simulink model "V2GCKT"  (R2016b)
settings: Solver=ode23t  StartTime=0.0  StopTime=1  RelTol=1e-3
undefined symbols (not defined in the file): Ion, Lithium
libraries: powerlib x27, powerlib_meascontrol x8, simulink x5, electricdrivelib x1
settings Model: Creator=acer  LastModifiedBy=acer

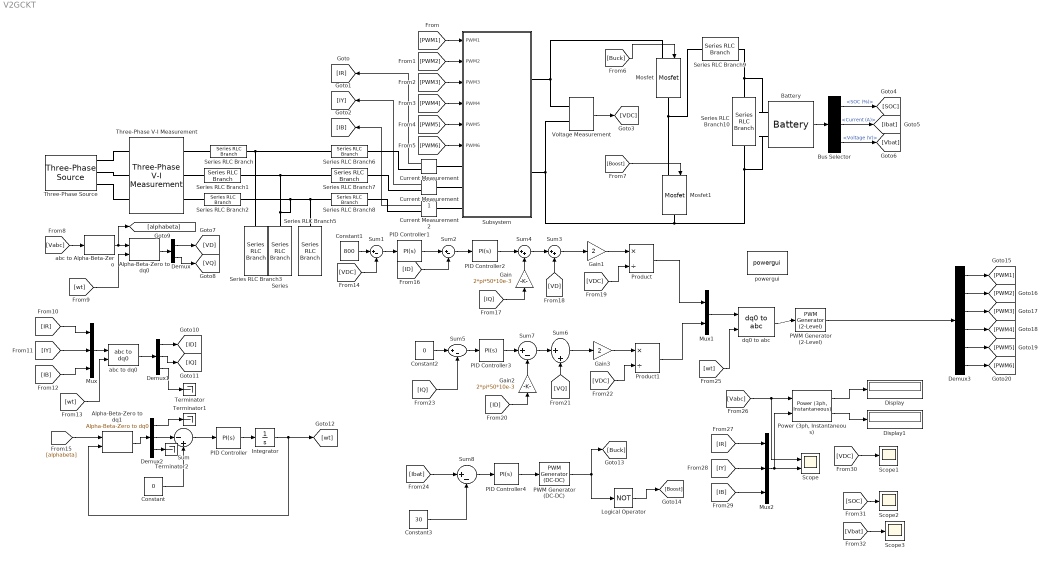
== system V2GCKT ==
  Alpha-Beta-Zero to dq0 : powerlib_meascontrol/Transformations/Alpha-Beta-Zero to dq0  Alignment=90 degrees behind phase A axis
  Alpha-Beta-Zero to dq1 : powerlib_meascontrol/Transformations/Alpha-Beta-Zero to dq0  Alignment=90 degrees behind phase A axis
  Battery : electricdrivelib/Extra Sources/Battery  BatType=Lithium-Ion  ShowTempParam=off  ThermalPreset=no  NomV=360  NomQ=300  SOC=50  Batt_Tr=1  PresetModel=on  MaxQ=300  MinV=270  FullV=419.0354  Dis_rate=130.4348  R=0.012  Normal_OP=271.3043  expZone="[388.9389      14.73913]"  current=[6.5 13 32.5]  Units=Time  Tci=20  NomT=25  T2=0  MaxQ2=2.208  FullV2=3.45  Normal_OP2=2.8  expZone2="[3.22        0.23]"  Rca=0.6  ti=1000  Dp=0
  Bus Selector : BusSelector  OutputSignals=SOC (%),Current (A),Voltage (V)
  Constant : Constant  Value=0
  Constant1 : Constant  Value=800
  Constant2 : Constant  Value=0
  Constant3 : Constant  Value=30
  Current Measurement : powerlib/Measurements/Current Measurement  PhasorSimulation=off  OutputType=Complex  PSBequivalent=0
  Current Measurement1 : powerlib/Measurements/Current Measurement  PhasorSimulation=off  OutputType=Complex  PSBequivalent=0
  Current Measurement2 : powerlib/Measurements/Current Measurement  PhasorSimulation=off  OutputType=Complex  PSBequivalent=0
  Demux : Demux  Outputs=2
  Demux1 : Demux  Outputs=3
  Demux2 : Demux  Outputs=3
  Demux3 : Demux  Outputs=6
  Display : Display
  Display1 : Display
  Gain : Gain  Gain=2*pi*50*10e-3
  Gain1 : Gain  Gain=2
  Gain2 : Gain  Gain=2*pi*50*10e-3
  Gain3 : Gain  Gain=2
  Integrator : Integrator
  Logical Operator : Logic  Operator=NOT  AllPortsSameDT=off  OutDataTypeStr=boolean
  Mosfet : powerlib/Power Electronics/Mosfet  Ron=0.1  Lon=0  Rd=0.01  Vfd=0  IC=0  Rs=1e5  Cs=inf  Measurements=off
  Mosfet1 : powerlib/Power Electronics/Mosfet  Ron=0.1  Lon=0  Rd=0.01  Vfd=0  IC=0  Rs=1e5  Cs=inf  Measurements=off
  Mux : Mux  Inputs=3
  Mux1 : Mux  Inputs=2
  Mux2 : Mux  Inputs=3
  PID Controller : simulink/Continuous/PID Controller  Controller=PI  TimeDomain=Continuous-time  SampleTime=-1  IntegratorMethod=Forward Euler  FilterMethod=Forward Euler  Form=Parallel  UseFilter=on  ControllerParametersSource=internal  P=10  I=50000  D=0  N=100  InitialConditionSource=internal  InitialConditionForIntegrator=0  InitialConditionForFilter=0  ExternalReset=none  LimitOutput=off  UpperSaturationLimit=inf  LowerSaturationLimit=-inf  LinearizeAsGain=on  AntiWindupMode=none  Kb=1  TrackingMode=off  Kt=1  PParamMin=[]  PParamMax=[]  IParamMin=[]  IParamMax=[]  DParamMin=[]  DParamMax=[]  NParamMin=[]  NParamMax=[]  KbParamMin=[]  KbParamMax=[]  KtParamMin=[]  KtParamMax=[]  POutMin=[]  POutMax=[]  IOutMin=[]  IOutMax=[]  DOutMin=[]  DOutMax=[]  NOutMin=[]  NOutMax=[]  KbOutMin=[]  KbOutMax=[]  KtOutMin=[]  KtOutMax=[]  IntegratorOutMin=[]  IntegratorOutMax=[]  FilterOutMin=[]  FilterOutMax=[]  SumOutMin=[]  SumOutMax=[]  SumI1OutMin=[]  SumI1OutMax=[]  SumI2OutMin=[]  SumI2OutMax=[]  SumI3OutMin=[]  SumI3OutMax=[]  SumDOutMin=[]  SumDOutMax=[]  SaturationOutMin=[]  SaturationOutMax=[]  IntegratorContinuousStateAttributes=''  IntegratorStateMustResolveToSignalObject=off  IntegratorRTWStateStorageClass=Auto  FilterContinuousStateAttributes=''  FilterStateMustResolveToSignalObject=off  FilterRTWStateStorageClass=Auto  DifferentiatorICPrevScaledInput=0  DifferentiatorOutMin=[]  DifferentiatorOutMax=[]
  PID Controller1 : simulink/Continuous/PID Controller  Controller=PI  TimeDomain=Continuous-time  SampleTime=-1  IntegratorMethod=Forward Euler  FilterMethod=Forward Euler  Form=Parallel  UseFilter=on  ControllerParametersSource=internal  P=0.5  I=5  D=0  N=100  InitialConditionSource=internal  InitialConditionForIntegrator=0  InitialConditionForFilter=0  ExternalReset=none  LimitOutput=off  UpperSaturationLimit=inf  LowerSaturationLimit=-inf  LinearizeAsGain=on  AntiWindupMode=none  Kb=1  TrackingMode=off  Kt=1  PParamMin=[]  PParamMax=[]  IParamMin=[]  IParamMax=[]  DParamMin=[]  DParamMax=[]  NParamMin=[]  NParamMax=[]  KbParamMin=[]  KbParamMax=[]  KtParamMin=[]  KtParamMax=[]  POutMin=[]  POutMax=[]  IOutMin=[]  IOutMax=[]  DOutMin=[]  DOutMax=[]  NOutMin=[]  NOutMax=[]  KbOutMin=[]  KbOutMax=[]  KtOutMin=[]  KtOutMax=[]  IntegratorOutMin=[]  IntegratorOutMax=[]  FilterOutMin=[]  FilterOutMax=[]  SumOutMin=[]  SumOutMax=[]  SumI1OutMin=[]  SumI1OutMax=[]  SumI2OutMin=[]  SumI2OutMax=[]  SumI3OutMin=[]  SumI3OutMax=[]  SumDOutMin=[]  SumDOutMax=[]  SaturationOutMin=[]  SaturationOutMax=[]  IntegratorContinuousStateAttributes=''  IntegratorStateMustResolveToSignalObject=off  IntegratorRTWStateStorageClass=Auto  FilterContinuousStateAttributes=''  FilterStateMustResolveToSignalObject=off  FilterRTWStateStorageClass=Auto  DifferentiatorICPrevScaledInput=0  DifferentiatorOutMin=[]  DifferentiatorOutMax=[]
  PID Controller2 : simulink/Continuous/PID Controller  Controller=PI  TimeDomain=Continuous-time  SampleTime=-1  IntegratorMethod=Forward Euler  FilterMethod=Forward Euler  Form=Parallel  UseFilter=on  ControllerParametersSource=internal  P=25  I=500  D=0  N=100  InitialConditionSource=internal  InitialConditionForIntegrator=0  InitialConditionForFilter=0  ExternalReset=none  LimitOutput=off  UpperSaturationLimit=inf  LowerSaturationLimit=-inf  LinearizeAsGain=on  AntiWindupMode=none  Kb=1  TrackingMode=off  Kt=1  PParamMin=[]  PParamMax=[]  IParamMin=[]  IParamMax=[]  DParamMin=[]  DParamMax=[]  NParamMin=[]  NParamMax=[]  KbParamMin=[]  KbParamMax=[]  KtParamMin=[]  KtParamMax=[]  POutMin=[]  POutMax=[]  IOutMin=[]  IOutMax=[]  DOutMin=[]  DOutMax=[]  NOutMin=[]  NOutMax=[]  KbOutMin=[]  KbOutMax=[]  KtOutMin=[]  KtOutMax=[]  IntegratorOutMin=[]  IntegratorOutMax=[]  FilterOutMin=[]  FilterOutMax=[]  SumOutMin=[]  SumOutMax=[]  SumI1OutMin=[]  SumI1OutMax=[]  SumI2OutMin=[]  SumI2OutMax=[]  SumI3OutMin=[]  SumI3OutMax=[]  SumDOutMin=[]  SumDOutMax=[]  SaturationOutMin=[]  SaturationOutMax=[]  IntegratorContinuousStateAttributes=''  IntegratorStateMustResolveToSignalObject=off  IntegratorRTWStateStorageClass=Auto  FilterContinuousStateAttributes=''  FilterStateMustResolveToSignalObject=off  FilterRTWStateStorageClass=Auto  DifferentiatorICPrevScaledInput=0  DifferentiatorOutMin=[]  DifferentiatorOutMax=[]
  PID Controller3 : simulink/Continuous/PID Controller  Controller=PI  TimeDomain=Continuous-time  SampleTime=-1  IntegratorMethod=Forward Euler  FilterMethod=Forward Euler  Form=Parallel  UseFilter=on  ControllerParametersSource=internal  P=25  I=500  D=0  N=100  InitialConditionSource=internal  InitialConditionForIntegrator=0  InitialConditionForFilter=0  ExternalReset=none  LimitOutput=off  UpperSaturationLimit=inf  LowerSaturationLimit=-inf  LinearizeAsGain=on  AntiWindupMode=none  Kb=1  TrackingMode=off  Kt=1  PParamMin=[]  PParamMax=[]  IParamMin=[]  IParamMax=[]  DParamMin=[]  DParamMax=[]  NParamMin=[]  NParamMax=[]  KbParamMin=[]  KbParamMax=[]  KtParamMin=[]  KtParamMax=[]  POutMin=[]  POutMax=[]  IOutMin=[]  IOutMax=[]  DOutMin=[]  DOutMax=[]  NOutMin=[]  NOutMax=[]  KbOutMin=[]  KbOutMax=[]  KtOutMin=[]  KtOutMax=[]  IntegratorOutMin=[]  IntegratorOutMax=[]  FilterOutMin=[]  FilterOutMax=[]  SumOutMin=[]  SumOutMax=[]  SumI1OutMin=[]  SumI1OutMax=[]  SumI2OutMin=[]  SumI2OutMax=[]  SumI3OutMin=[]  SumI3OutMax=[]  SumDOutMin=[]  SumDOutMax=[]  SaturationOutMin=[]  SaturationOutMax=[]  IntegratorContinuousStateAttributes=''  IntegratorStateMustResolveToSignalObject=off  IntegratorRTWStateStorageClass=Auto  FilterContinuousStateAttributes=''  FilterStateMustResolveToSignalObject=off  FilterRTWStateStorageClass=Auto  DifferentiatorICPrevScaledInput=0  DifferentiatorOutMin=[]  DifferentiatorOutMax=[]
  PID Controller4 : simulink/Continuous/PID Controller  Controller=PI  TimeDomain=Continuous-time  SampleTime=-1  IntegratorMethod=Forward Euler  FilterMethod=Forward Euler  Form=Parallel  UseFilter=on  ControllerParametersSource=internal  P=0.005  I=10  D=0  N=100  InitialConditionSource=internal  InitialConditionForIntegrator=0  InitialConditionForFilter=0  ExternalReset=none  LimitOutput=on  UpperSaturationLimit=0.95  LowerSaturationLimit=0  LinearizeAsGain=on  AntiWindupMode=none  Kb=1  TrackingMode=off  Kt=1  PParamMin=[]  PParamMax=[]  IParamMin=[]  IParamMax=[]  DParamMin=[]  DParamMax=[]  NParamMin=[]  NParamMax=[]  KbParamMin=[]  KbParamMax=[]  KtParamMin=[]  KtParamMax=[]  POutMin=[]  POutMax=[]  IOutMin=[]  IOutMax=[]  DOutMin=[]  DOutMax=[]  NOutMin=[]  NOutMax=[]  KbOutMin=[]  KbOutMax=[]  KtOutMin=[]  KtOutMax=[]  IntegratorOutMin=[]  IntegratorOutMax=[]  FilterOutMin=[]  FilterOutMax=[]  SumOutMin=[]  SumOutMax=[]  SumI1OutMin=[]  SumI1OutMax=[]  SumI2OutMin=[]  SumI2OutMax=[]  SumI3OutMin=[]  SumI3OutMax=[]  SumDOutMin=[]  SumDOutMax=[]  SaturationOutMin=[]  SaturationOutMax=[]  IntegratorContinuousStateAttributes=''  IntegratorStateMustResolveToSignalObject=off  IntegratorRTWStateStorageClass=Auto  FilterContinuousStateAttributes=''  FilterStateMustResolveToSignalObject=off  FilterRTWStateStorageClass=Auto  DifferentiatorICPrevScaledInput=0  DifferentiatorOutMin=[]  DifferentiatorOutMax=[]
  PWM Generator (2-Level) : powerlib_meascontrol/Pulse & Signal Generators/PWM Generator (2-Level)  ModulatorType=Three-phase bridge (6 pulses)  ModulatorMode=Unsynchronized  Fc=10000  Pc=90  nF=27  MinMax="[ -1  1 ]"  SamplingTechnique=Natural  ModulatingSignals=off  m=0.8  Freq=60  Phase=0  Ts=0  ShowCarrierOutport=off
  PWM Generator (DC-DC) : powerlib_meascontrol/Pulse & Signal Generators/PWM Generator (DC-DC)  Fsw=10000  Ts=0
  "Power (3ph, Instantaneous)" : powerlib_meascontrol/Measurements/Power (3ph, Instantaneous)
  Product : Product  Inputs=*/
  Product1 : Product  Inputs=*/
  Scope : Scope  NumInputPorts=2
  Scope1 : Scope
  Scope2 : Scope
  Scope3 : Scope
  "Series " : powerlib/Elements/Series RLC Branch  LConnTagsString=__new0  RConnTagsString=__new0  BranchType=C  Resistance=1  Inductance=1e-3  SetiL0=off  InitialCurrent=0  Capacitance=30e-6  Setx0=off  InitialVoltage=0  Measurements=None
  Series RLC Branch{,1..2,6..8} (6 alike) : powerlib/Elements/Series RLC Branch  LConnTagsString=__new0  RConnTagsString=__new0  BranchType=L  Resistance=1  Inductance=5e-3  SetiL0=off  InitialCurrent=0  Capacitance=1e-6  Setx0=off  InitialVoltage=0  Measurements=None
  Series RLC Branch10 : powerlib/Elements/Series RLC Branch  LConnTagsString=__new0  RConnTagsString=__new0  BranchType=RC  Resistance=0.0001  Inductance=20e-3  SetiL0=off  InitialCurrent=0  Capacitance=0.625e-6  Setx0=off  InitialVoltage=0  Measurements=None
  Series RLC Branch3 : powerlib/Elements/Series RLC Branch  LConnTagsString=__new0  RConnTagsString=__new0  BranchType=C  Resistance=1  Inductance=1e-3  SetiL0=off  InitialCurrent=0  Capacitance=30e-6  Setx0=off  InitialVoltage=0  Measurements=None
  Series RLC Branch5 : powerlib/Elements/Series RLC Branch  LConnTagsString=__new0  RConnTagsString=__new0  BranchType=C  Resistance=1  Inductance=1e-3  SetiL0=off  InitialCurrent=0  Capacitance=30e-6  Setx0=off  InitialVoltage=0  Measurements=None
  Series RLC Branch9 : powerlib/Elements/Series RLC Branch  LConnTagsString=__new0  RConnTagsString=__new0  BranchType=RL  Resistance=0.0001  Inductance=20e-3  SetiL0=off  InitialCurrent=0  Capacitance=1e-6  Setx0=off  InitialVoltage=0  Measurements=None
  Subsystem : Subsystem
  Sum : Sum  Inputs=|-+
  Sum{1..2,5,7..8} (5 alike) : Sum  Inputs=|+-
  Sum3 : Sum  Inputs=|++
  Sum4 : Sum  Inputs=|++
  Sum6 : Sum  Inputs=|++
  Terminator : Terminator
  Terminator1 : Terminator
  Terminator2 : Terminator
  Three-Phase V-I Measurement : powerlib/Measurements/Three-Phase V-I Measurement  VoltageMeasurement=phase-to-ground  SetLabelV=on  LabelV=Vabc  Vpu=off  VpuLL=off  CurrentMeasurement=no  SetLabelI=off  LabelI=Iabc  Ipu=off  Pbase=100e6  Vbase=500e3  OutputType=Complex  PhasorSimulation=off  PSBequivalent=0
  Three-Phase Source : powerlib/Electrical Sources/Three-Phase Source  InternalConnection=Yg  VoltagePhases=off  Voltage=415  PhaseAngle=0  Voltage_phases=[25e3 25e3 25e3]/sqrt(3)  PhaseAngles_phases=[0 -120 +120]  Frequency=50  NonIdealSource=on  SpecifyImpedance=off  Resistance=0.8929e-3  Inductance=16.58e-9  ShortCircuitLevel=100e6  BaseVoltage=415  XRratio=7  BusType=swing  Pref=10e3  Qref=0  Prefabc=[10e3, 10e3, 10e3]  Qrefabc=[0, 0, 0]  Qmin=-inf  Qmax=inf
  Voltage Measurement : powerlib/Measurements/Voltage Measurement  PhasorSimulation=off  OutputType=Complex  PSBequivalent=0
  abc to Alpha-Beta-Zero : powerlib_meascontrol/Transformations/abc to Alpha-Beta-Zero
  abc to dq0 : powerlib_meascontrol/Transformations/abc to dq0  Alignment=90 degrees behind phase A axis
  dq0 to abc : powerlib_meascontrol/Transformations/dq0 to abc  Alignment=90 degrees behind phase A axis
  powergui : powerlib/powergui  Priority=1  SimulationMode=Discrete  SolverType=Tustin/Backward Euler (TBE)  SampleTime=1e-6  frequency=60  SPID=off  DisableSnubberDevices=off  DisableRonSwitches=off  DisableVfSwitches=off  SwTol=0  DisplayEquations=off  Interpol=off  ExternalGateDelay=off  methode=off  Ts=10  FunctionMessages=off  echomessages=off  HookPort=off  EnableUseOfTLC=off  x0status=blocks  frequencyindice=50  Pbase=100e6  ErrMax=1e-4  Iterations=50  UnitsV=kV  UnitsW=MW  buscounter=0  RestoreLinks=warning  ResistiveCurrentMeasurement=off  Frange=[0:2:500]  Ylog=off  Xlog=on  ShowGrid=off  save=off  variable=ZData  structure=0  ZoomFFT=off  StartTime=0.0  cycles=1  DisplayStyle=1  fundamental=60  FreqAxis=off  MaxFrequency=1000  frequencyindicesteady=1  RmsSteady=1  display=off
  wires:
  [PWM1] -> Subsystem/1(PWM1)
  [PWM2] -> Subsystem/2(PWM2)
  [PWM3] -> Subsystem/3(PWM3)
  [PWM4] -> Subsystem/4(PWM4)
  [PWM5] -> Subsystem/5(PWM5)
  [PWM6] -> Subsystem/6(PWM6)
  Voltage Measurement/1 -> [VDC]
  [Buck] -> Mosfet/1
  [Boost] -> Mosfet1/1
  Battery/1 -> Bus Selector/1
  [Vabc] -> abc to Alpha-Beta-Zero/1
  abc to Alpha-Beta-Zero/1 -> [alphabeta], Alpha-Beta-Zero to dq0/1
  Alpha-Beta-Zero to dq0/1 -> Demux/1
  Demux/1 -> [VD]
  Demux/2 -> [VQ]
  Mux/1 -> abc to dq0/1
  [wt] -> abc to dq0/2
  abc to dq0/1 -> Demux1/1
  [alphabeta] -> Alpha-Beta-Zero to dq1/1
  [IR] -> Mux/1
  [IY] -> Mux/2
  [IB] -> Mux/3
  Alpha-Beta-Zero to dq1/1 -> Demux2/1
  Constant/1 -> Sum/2
  Sum/1 -> PID Controller/1
  PID Controller/1 -> Integrator/1
  Integrator/1 -> [wt], Alpha-Beta-Zero to dq1/2
  Constant1/1 -> Sum1/1
  [VDC] -> Sum1/2
  Sum1/1 -> PID Controller1/1
  PID Controller1/1 -> Sum2/1
  [ID] -> Sum2/2
  Sum2/1 -> PID Controller2/1
  PID Controller2/1 -> Sum4/1
  Gain/1 -> Sum4/2
  [IQ] -> Gain/1
  Sum4/1 -> Sum3/1
  [VD] -> Sum3/2
  Sum3/1 -> Gain1/1
  Gain1/1 -> Product/1
  [VDC] -> Product/2
  Sum5/1 -> PID Controller3/1
  PID Controller3/1 -> Sum7/1
  Gain2/1 -> Sum7/2
  [ID] -> Gain2/1
  Sum7/1 -> Sum6/1
  [VQ] -> Sum6/2
  Sum6/1 -> Gain3/1
  Gain3/1 -> Product1/1
  [VDC] -> Product1/2
  Constant2/1 -> Sum5/1
  [IQ] -> Sum5/2
  [Ibat] -> Sum8/1
  Constant3/1 -> Sum8/2
  Sum8/1 -> PID Controller4/1
  PID Controller4/1 -> PWM Generator (DC-DC)/1
  PWM Generator (DC-DC)/1 -> Logical Operator/1, [Buck]
  Logical Operator/1 -> [Boost]
  [wt] -> dq0 to abc/2
  dq0 to abc/1 -> PWM Generator (2-Level)/1
  PWM Generator (2-Level)/1 -> Demux3/1
  Demux3/1 -> [PWM1]
  Demux3/2 -> [PWM2]
  Demux3/3 -> [PWM3]
  Demux3/4 -> [PWM4]
  Demux3/5 -> [PWM5]
  Demux3/6 -> [PWM6]
  [Vabc] -> Scope/1, "Power (3ph, Instantaneous)"/1
  [IR] -> Mux2/1
  [IY] -> Mux2/2
  [IB] -> Mux2/3
  Mux2/1 -> Scope/2, "Power (3ph, Instantaneous)"/2
  [VDC] -> Scope1/1
  "Power (3ph, Instantaneous)"/2 -> Display1/1
  Current Measurement/1 -> [IR]
  Current Measurement1/1 -> [IY]
  Current Measurement2/1 -> [IB]
  Bus Selector/1 -> [SOC]  "<SOC (%)>"
  Mux1/1 -> dq0 to abc/1
  Product1/1 -> Mux1/2
  Product/1 -> Mux1/1
  Bus Selector/3 -> [Vbat]  "<Voltage (V)>"
  Bus Selector/2 -> [Ibat]  "<Current (A)>"
  [SOC] -> Scope2/1
  [Vbat] -> Scope3/1
  [wt] -> Alpha-Beta-Zero to dq0/2
  Demux2/2 -> Sum/1
  Demux1/1 -> [ID]
  Demux1/2 -> [IQ]
  Demux1/3 -> Terminator/1
  Demux2/1 -> Terminator1/1
  Demux2/3 -> Terminator2/1
  "Power (3ph, Instantaneous)"/1 -> Display/1
  connections:
  Three-Phase V-I Measurement/LConn2 -- Three-Phase Source/RConn2
  Three-Phase V-I Measurement/LConn3 -- Three-Phase Source/RConn3
  Three-Phase V-I Measurement/LConn1 -- Three-Phase Source/RConn1
  Series RLC Branch/LConn1 -- Three-Phase V-I Measurement/RConn1
  Series RLC Branch1/LConn1 -- Three-Phase V-I Measurement/RConn2
  Series RLC Branch2/LConn1 -- Three-Phase V-I Measurement/RConn3
  Series RLC Branch/RConn1 -- Series RLC Branch6/LConn1 -- Series RLC Branch3/LConn1
  Series RLC Branch5/LConn1 -- Series RLC Branch8/LConn1 -- "Series "/LConn1 -- Series RLC Branch1/RConn1 -- Series RLC Branch7/LConn1 -- Series RLC Branch2/RConn1
  Voltage Measurement/LConn2 -- Battery/LConn2 -- Series RLC Branch10/RConn1 -- Mosfet1/RConn1 -- Subsystem/RConn2
  Voltage Measurement/LConn1 -- Mosfet/LConn1 -- Subsystem/RConn1
  Mosfet1/LConn1 -- Series RLC Branch9/LConn1 -- Mosfet/RConn1
  Series RLC Branch10/LConn1 -- Battery/LConn1 -- Series RLC Branch9/RConn1
  Current Measurement/LConn1 -- Subsystem/LConn1
  Current Measurement1/LConn1 -- Subsystem/LConn2
  Current Measurement2/LConn1 -- Subsystem/LConn3
  Series RLC Branch6/RConn1 -- Current Measurement/RConn1
  Series RLC Branch7/RConn1 -- Current Measurement1/RConn1
  Series RLC Branch8/RConn1 -- Current Measurement2/RConn1

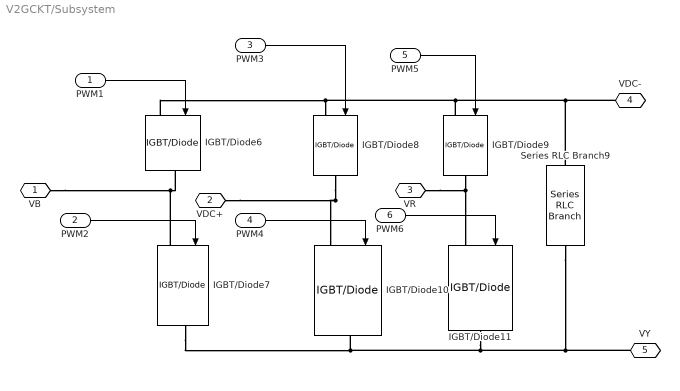
== system V2GCKT/Subsystem ==
  PWM1 : Inport
  PWM2 : Inport  Port=2
  PWM3 : Inport  Port=3
  PWM4 : Inport  Port=4
  PWM5 : Inport  Port=5
  PWM6 : Inport  Port=6
  IGBT/Diode{6..11} (6 alike) : powerlib/Power Electronics/IGBT//Diode  Ron=1e-3  Rs=1e5  Cs=inf  Measurements=off
  Series RLC Branch9 : powerlib/Elements/Series RLC Branch  LConnTagsString=__new0  RConnTagsString=__new0  BranchType=RC  Resistance=1e-3  Inductance=1e-3  SetiL0=off  InitialCurrent=0  Capacitance=5600e-6  Setx0=on  InitialVoltage=800  Measurements=None
  VB : PMIOPort  Port=1  Side=Left
  VDC+ : PMIOPort  Port=2  Side=Right
  VR : PMIOPort  Port=3  Side=Left
  VDC- : PMIOPort  Port=4  Side=Right
  VY : PMIOPort  Port=5  Side=Left
  wires:
  PWM2/1 -> IGBT/Diode7/1
  PWM5/1 -> IGBT/Diode9/1
  PWM6/1 -> IGBT/Diode11/1
  PWM3/1 -> IGBT/Diode8/1
  PWM4/1 -> IGBT/Diode10/1
  PWM1/1 -> IGBT/Diode6/1
  connections:
  IGBT/Diode6/LConn1 -- VDC-/RConn1 -- Series RLC Branch9/LConn1 -- IGBT/Diode9/LConn1 -- IGBT/Diode8/LConn1
  IGBT/Diode7/RConn1 -- VY/RConn1 -- Series RLC Branch9/RConn1 -- IGBT/Diode11/RConn1 -- IGBT/Diode10/RConn1
  IGBT/Diode8/RConn1 -- VDC+/RConn1 -- IGBT/Diode10/LConn1
  IGBT/Diode7/LConn1 -- VB/RConn1 -- IGBT/Diode6/RConn1
  IGBT/Diode9/RConn1 -- VR/RConn1 -- IGBT/Diode11/LConn1
